simulink model "mechanicalDLTorsionOrderMap"  (R2025b)
settings: Solver=ode1be  StartTime=0.0  StopTime=5  FixedStep=0.001  RelTol=1e-3
PreLoadFcn:
  | mechanicalDLTorsionOrderMapParams;
undefined symbols (not defined in the file): mechDLParams
libraries: fl_lib x24, nesl_utility x4
settings Model: Creator=shachind  LastModifiedBy=shachind
settings SimscapeCC: SimscapeLogType=all  SimscapeLogName=simlogMechanicalDLTorsion  SimscapeLogLimitData=off

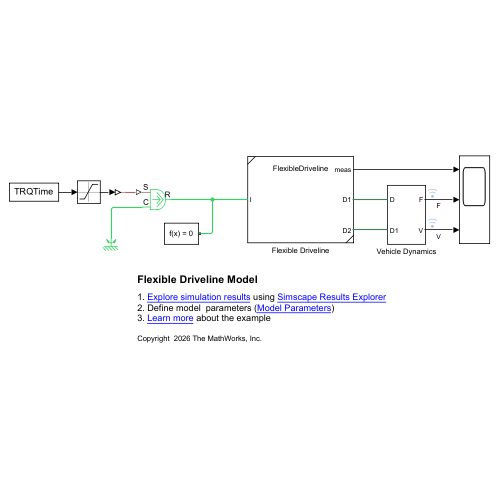
[thumbnail: Simulink's stored preview of the top-level diagram]
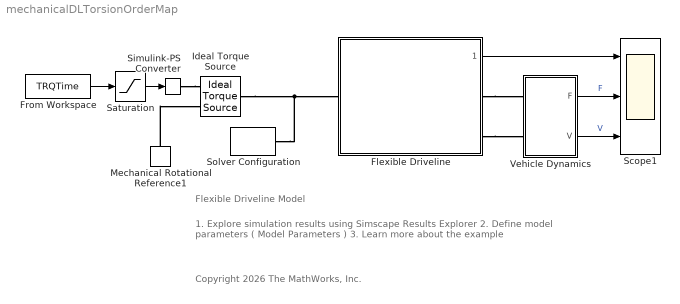
== system mechanicalDLTorsionOrderMap ==
  note: Copyright 2026 The MathWorks, Inc.
  note: Flexible Driveline Model
  note: 1. Explore simulation results using Simscape Results Explorer
      | 2. Define model parameters ( Model Parameters )
      | 3. Learn more about the example
  Flexible Driveline : Subsystem  ReferencedSubsystem=FlexibleDriveline
  From Workspace : FromWorkspace  VariableName=TRQTime  OutputAfterFinalValue=Holding final value
  Ideal Torque Source : fl_lib/Mechanical/Mechanical Sources/Ideal Torque Source
  Mechanical Rotational Reference1 : fl_lib/Mechanical/Rotational Elements/Mechanical Rotational Reference
  Saturation : Saturate  UpperLimit=inf  LowerLimit=0
  Scope1 : Scope  NumInputPorts=3
      settings: ShowGrid=off  ActiveDisplayYMinimum=-125.91158915677352  ActiveDisplayYMaximum=877.36348223231357
  Simulink-PS Converter : nesl_utility/Simulink-PS Converter  PhysicalDomain=network_engine_domain  SubClassName=ps_input  LeftPortType=input  RightPortType=output  PseudoPeriodic=off  Frequencies=[]  NoiseDistribution=none  NoiseParameters=[]  Unit=1  AffineConversion=off  FilteringAndDerivatives=provide  SimscapeFilterOrder=1  InputFilterTimeConstant=0.001  UdotUserProvided=0
  Solver Configuration : nesl_utility/Solver Configuration  PhysicalDomain=network_engine_domain  SubClassName=solver  LeftPortType=input  RightPortType=generic  Tones=[]  Harmonics=[]  SimulateNoise=off  Profile=off  UseLocalSampling=off  EnableSwitchedLinearOptims=on  FrequencyDomain=off  UseCCode=off  RelTol=0.001  AbsTol=0.001  MinStep=1e-09  ToWorkspace=off  RevertToSquareIcSolve=off  NumHomotopyIterations=100  PhasorMode=off  PhasorModeNumHarmonics=1  ConsistencySolver=NEWTON_XTOL_AFTER_FTOL  IndexReductionMethod=DerivativeReplacement  DoDC=off  ResidualTolerance=1e-09  ConsistencyTolSource=GLOBAL  ConsistencyAbsTol=0.001  ConsistencyRelTol=0.001  ConsistencyTolFactor=0.001  UseLocalSolver=on  LocalSolverChoice=NE_BACKWARD_EULER_ADVANCER  ResolveIndetEquations=on  FunctionEvalNumThread=1  LocalSolverSampleTime=0.001  DoFixedCost=off  MaxNonlinIter=3  MaxModeIter=2  ComputeImpulses=off  ImpulseIterations=2  LinearAlgebra=auto  LinearAlgebraNumThread=0  EquationFormulation=NE_TIME_EF  DelaysMemoryBudget=1024  AutomaticFiltering=on  FilteringTimeConstant=0.001  PartitionStorageMethod=AS_NEEDED  PartitionMemoryBudget=1024  PartitionMethod=ROBUST  MultibodyUseLocalSolver=off  MultibodyLocalSolverChoice=ODE1  MultibodyLocalSolverSampleTime=0.001
  Vehicle Dynamics : Subsystem
  wires:
  From Workspace/1 -> Saturation/1
  Flexible Driveline/1 -> Scope1/1
  Saturation/1 -> Simulink-PS Converter/1
  Vehicle Dynamics/1(F) -> Scope1/2  "F"
  Vehicle Dynamics/2(V) -> Scope1/3  "V"
  connections:
  Flexible Driveline/RConn1 -- Vehicle Dynamics/LConn1
  Ideal Torque Source/LConn1 -- Solver Configuration/RConn1 -- Flexible Driveline/LConn1
  Simulink-PS Converter/RConn1 -- Ideal Torque Source/RConn1
  Mechanical Rotational Reference1/LConn1 -- Ideal Torque Source/RConn2
  Flexible Driveline/RConn2 -- Vehicle Dynamics/LConn2

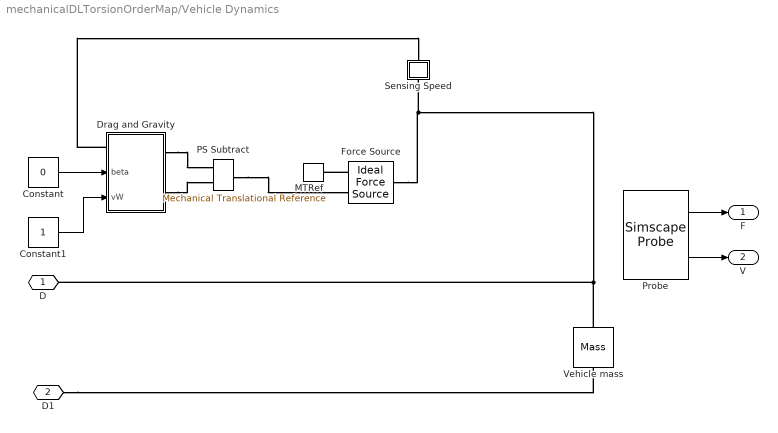
== system mechanicalDLTorsionOrderMap/Vehicle Dynamics ==
  Constant : Constant  Value=0
  Constant1 : Constant
  Drag and Gravity : Subsystem
      settings: PortSchema="{\"entries\":[{\"content\":{\"sides\":[{\"content\":{\"connectorIds\":[\"LConn1\",\"In1\",\"In2\"]},\"type\":\"ConnectorPlacement.EquallySpacedRectSide\",\"uuid\":\"54aa6f83-5d7e-47eb-af0d-7f3161a8ff41\"},{\"content\":{\"connectorIds\":[\"RConn1\",\"RConn2\"],\"side\":\"RIGHT\"},\"type\":\"ConnectorPlacement.EquallySpacedRectSide\",\"uuid\":\"b4f0cef7-4bdf-4dc5-a509-752bd08bffb1\"},{\"content\":{\"side\":\"TOP\"},\"type\":\"ConnectorPlacement.EquallySpacedRectSide\",\"uuid\":\"5d5d0916-3855-4ad3-a369-cf767cdced70\"}]},\"type\":\"ConnectorPlacement.EquallySpacedConnector\",\"uuid\":\"79a1b4b7-87bd-4fe6-ab94-84f266f33e3e\"}],\"packageUris\":[\"http://schema.mathworks.com/mf0/Connector/R2020b\"],\"version\":\"1.0\"}"
  Force Source : fl_lib/Mechanical/Mechanical Sources/Ideal Force Source
  MTRef : fl_lib/Mechanical/Translational Elements/Mechanical Translational Reference
  PS Subtract : fl_lib/Physical Signals/Functions/PS Subtract
  Probe : SimscapeProbe  BoundBlock=50  Variables="{\"f\":{\"Probing\":\"ON\"},\"v\":{\"Unit\":\"mph\",\"Probing\":\"ON\"}}"
  Sensing Speed : Subsystem
      mask Display: disp('v')
  Vehicle mass : fl_lib/Mechanical/Translational Elements/Mass  mass=mechDLParams.vehicle.mass kg  num_ports=foundation.enum.numPorts2.two  v_specify=off  v_priority=High  v=0 m/s  v_nominal_specify=off  v_nominal_value=1  v_nominal_unit=m/s  f_specify=off  f_priority=None  f=0 N  f_nominal_specify=off  f_nominal_value=1  f_nominal_unit=N
      settings: InternalSimscapePortConfiguration="{\"Bottom\":[],\"Left\":[{\"id\":\"M\",\"label\":\"\",\"type\":\"foundation.mechanical.translational.translational\"}],\"Right\":[{\"id\":\"N\",\"label\":\"\",\"type\":\"foundation.mechanical.translational.translational\"}],\"Top\":[]}"
  D : PMIOPort  Side=Left
  D1 : PMIOPort  Port=2  Side=Left
  F : Outport
  V : Outport  Port=2
  wires:
  Probe/1 -> F/1
  Constant/1 -> Drag and Gravity/1(beta)
  Constant1/1 -> Drag and Gravity/2(vW)
  Probe/2 -> V/1
  connections:
  Force Source/LConn1 -- Vehicle mass/LConn1 -- D/RConn1 -- Sensing Speed/LConn1
  D1/RConn1 -- Vehicle mass/RConn1
  Force Source/RConn2 -- MTRef/LConn1
  PS Subtract/RConn1 -- Force Source/RConn1
  Drag and Gravity/RConn1 -- PS Subtract/LConn1
  Drag and Gravity/RConn2 -- PS Subtract/LConn2
  Drag and Gravity/LConn1 -- Sensing Speed/RConn1

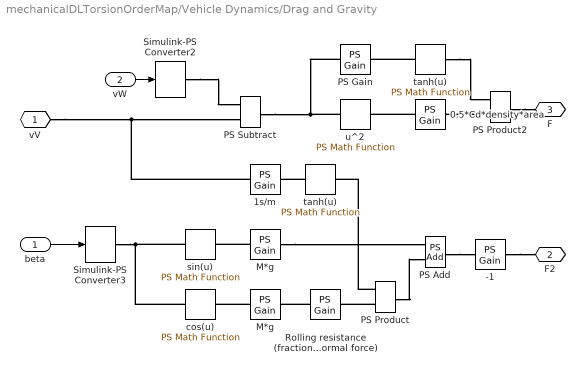
== system mechanicalDLTorsionOrderMap/Vehicle Dynamics/Drag and Gravity ==
  beta : Inport
  vW : Inport  Port=2
  " M*g " : fl_lib/Physical Signals/Functions/PS Gain  gain=mechDLParams.vehicle.mass*mechDLParams.vehicle.gravity kg*m/s^2
  " tanh(u) " : fl_lib/Physical Signals/Functions/PS Math Function  fcn_choice=foundation.enum.math_function.tanh  v=1
  -1 : fl_lib/Physical Signals/Functions/PS Gain  gain=-1
  0.5*Cd*density*area : fl_lib/Physical Signals/Functions/PS Gain  gain=0.5*mechDLParams.vehicle.dragCoefficient*mechDLParams.vehicle.airDensity*mechDLParams.vehicle.frontalArea kg/m^3*m^2
  1s/m : fl_lib/Physical Signals/Functions/PS Gain  gain=1 1/(m/s)
  M*g : fl_lib/Physical Signals/Functions/PS Gain  gain=mechDLParams.vehicle.mass*mechDLParams.vehicle.gravity kg*m/s^2
  PS Add : fl_lib/Physical Signals/Functions/PS Add
  PS Gain : fl_lib/Physical Signals/Functions/PS Gain  gain=1 1/(m/s)
  PS Product : fl_lib/Physical Signals/Functions/PS Product
  PS Product2 : fl_lib/Physical Signals/Functions/PS Product
  PS Subtract : fl_lib/Physical Signals/Functions/PS Subtract
  Rolling resistance (fraction of normal force) : fl_lib/Physical Signals/Functions/PS Gain  gain=mechDLParams.vehicle.tireRollingFriction
  Simulink-PS Converter2 : nesl_utility/Simulink-PS Converter  PhysicalDomain=network_engine_domain  SubClassName=ps_input  LeftPortType=input  RightPortType=output  PseudoPeriodic=off  Frequencies=[]  NoiseDistribution=none  NoiseParameters=[]  Unit=m/s  AffineConversion=off  FilteringAndDerivatives=zero  SimscapeFilterOrder=1  InputFilterTimeConstant=0.001  UdotUserProvided=1
  Simulink-PS Converter3 : nesl_utility/Simulink-PS Converter  PhysicalDomain=network_engine_domain  SubClassName=ps_input  LeftPortType=input  RightPortType=output  PseudoPeriodic=off  Frequencies=[]  NoiseDistribution=none  NoiseParameters=[]  Unit=deg  AffineConversion=off  FilteringAndDerivatives=zero  SimscapeFilterOrder=1  InputFilterTimeConstant=0.001  UdotUserProvided=1
  cos(u) : fl_lib/Physical Signals/Functions/PS Math Function  fcn_choice=foundation.enum.math_function.cos  v=1
  sin(u) : fl_lib/Physical Signals/Functions/PS Math Function  fcn_choice=foundation.enum.math_function.sin  v=1
  tanh(u) : fl_lib/Physical Signals/Functions/PS Math Function  fcn_choice=foundation.enum.math_function.tanh  v=1
  u^2 : fl_lib/Physical Signals/Functions/PS Math Function  fcn_choice=foundation.enum.math_function.square  v=1
  vV : PMIOPort  Side=Left
  F2 : PMIOPort  Port=2  Side=Right
  F : PMIOPort  Port=3  Side=Right
  wires:
  vW/1 -> Simulink-PS Converter2/1
  beta/1 -> Simulink-PS Converter3/1
  connections:
  vV/RConn1 -- 1s/m/LConn1 -- PS Subtract/LConn1
  Simulink-PS Converter2/RConn1 -- PS Subtract/LConn2
  PS Product2/RConn1 -- F/RConn1
  PS Product/LConn2 -- Rolling resistance (fraction of normal force)/RConn1
  PS Product/RConn1 -- PS Add/LConn2
  PS Add/RConn1 -- -1/LConn1
  -1/RConn1 -- F2/RConn1
  PS Product/LConn1 -- tanh(u)/RConn1
  tanh(u)/LConn1 -- 1s/m/RConn1
  PS Gain/LConn1 -- PS Subtract/RConn1 -- u^2/LConn1
  " tanh(u) "/RConn1 -- PS Product2/LConn1
  0.5*Cd*density*area/LConn1 -- u^2/RConn1
  " tanh(u) "/LConn1 -- PS Gain/RConn1
  PS Product2/LConn2 -- 0.5*Cd*density*area/RConn1
  cos(u)/LConn1 -- sin(u)/LConn1 -- Simulink-PS Converter3/RConn1
  M*g/RConn1 -- PS Add/LConn1
  Rolling resistance (fraction of normal force)/LConn1 -- " M*g "/RConn1
  M*g/LConn1 -- sin(u)/RConn1
  " M*g "/LConn1 -- cos(u)/RConn1

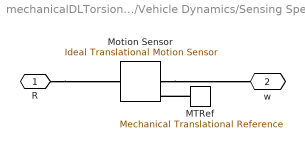
== system mechanicalDLTorsionOrderMap/Vehicle Dynamics/Sensing Speed ==
  MTRef : fl_lib/Mechanical/Translational Elements/Mechanical Translational Reference
  Motion Sensor : fl_lib/Mechanical/Mechanical Sensors/Ideal Translational Motion Sensor  reference=foundation.enum.MeasurementReference.difference  acceleration_port=false  velocity_port=true  position_port=true  offset=0 m
  R : PMIOPort  Side=Left
  w : PMIOPort  Port=2  Side=Right
  connections:
  Motion Sensor/RConn2 -- w/RConn1
  MTRef/LConn1 -- Motion Sensor/RConn1
  R/RConn1 -- Motion Sensor/LConn1
